simulink model "QuadArchitecture_AI"  (R2026b)
settings: Solver=ode4  StopTime=90  FixedStep=0.005
InitFcn:
  | init_stage02
settings Model: DataDictionary=QuadInterfaces_AI.sldd  Creator=JonathanTee  LastModifiedBy=JonathanTee

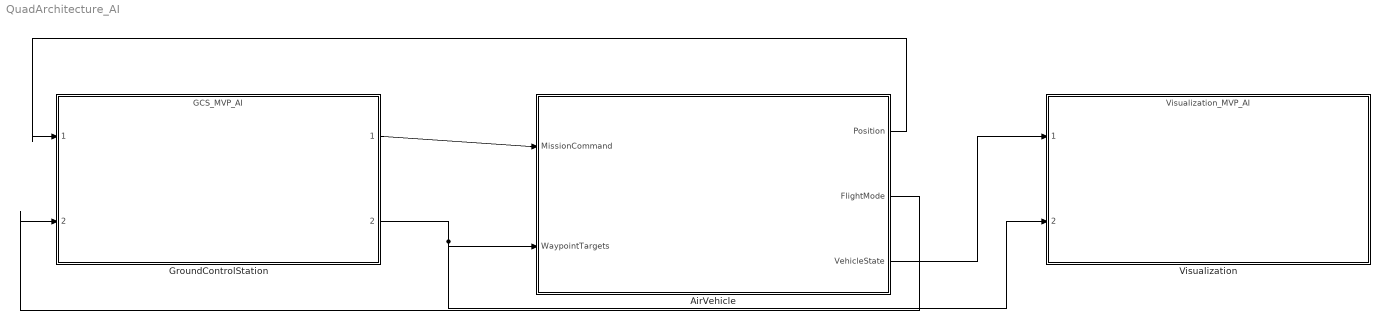
== system QuadArchitecture_AI ==
  AirVehicle : Subsystem
      settings: PortSchema="{\"entries\":[{\"content\":{\"headerSize\":26,\"margin\":15,\"minimumSpacing\":25,\"sides\":[{\"content\":{\"connectorIds\":[\"In1\",\"In2\"]},\"type\":\"ConnectorPlacement.EquallySpacedRectSide\",\"uuid\":\"ecfb2a5d-ebc3-4605-9a84-c6fd342510eb\"},{\"content\":{\"connectorIds\":[\"Out1\",\"Out2\",\"Out3\"],\"side\":\"RIGHT\"},\"type\":\"ConnectorPlacement.EquallySpacedRectSide\",\"uuid\":\"41ea779c-ccae-40c9-bf4c-62eb2a12d4ec\"},{\"content\":{\"side\":\"TOP\"},\"type\":\"ConnectorPlacement.EquallySpacedRectSide\",\"uuid\":\"f1fc56fa-babc-4d23-97d2-f02afcdd55d8\"}]},\"type\":\"ConnectorPlacement.EquallySpacedConnector\",\"uuid\":\"2007e49f-3d37-456e-85ff-e7f0d83353ae\"}],\"packageUris\":[\"http://schema.mathworks.com/mf0/Connector/R2020b\"],\"version\":\"1.0\"}"
  GroundControlStation : ModelReference  ModelNameDialog=GCS_MVP_AI  SimulationMode=Normal  ModelReferenceVersion=1.3
      settings: PortSchema="{\"entries\":[{\"content\":{\"headerSize\":38,\"margin\":15,\"minimumSpacing\":25,\"sides\":[{\"content\":{\"connectorIds\":[\"In1\",\"In2\"]},\"type\":\"ConnectorPlacement.EquallySpacedRectSide\",\"uuid\":\"ecfb2a5d-ebc3-4605-9a84-c6fd342510eb\"},{\"content\":{\"connectorIds\":[\"Out1\",\"Out2\"],\"side\":\"RIGHT\"},\"type\":\"ConnectorPlacement.EquallySpacedRectSide\",\"uuid\":\"41ea779c-ccae-40c9-bf4c-62eb2a12d4ec\"},{\"content\":{\"side\":\"TOP\"},\"type\":\"ConnectorPlacement.EquallySpacedRectSide\",\"uuid\":\"f1fc56fa-babc-4d23-97d2-f02afcdd55d8\"}]},\"type\":\"ConnectorPlacement.EquallySpacedConnector\",\"uuid\":\"2007e49f-3d37-456e-85ff-e7f0d83353ae\"}],\"packageUris\":[\"http://schema.mathworks.com/mf0/Connector/R2020b\"],\"version\":\"1.0\"}"
  Visualization : ModelReference  ModelNameDialog=Visualization_MVP_AI  SimulationMode=Normal  ModelReferenceVersion=1.2
      settings: PortSchema="{\"entries\":[{\"content\":{\"headerSize\":38,\"margin\":15,\"minimumSpacing\":25,\"sides\":[{\"content\":{\"connectorIds\":[\"In1\",\"In2\"]},\"type\":\"ConnectorPlacement.EquallySpacedRectSide\",\"uuid\":\"ecfb2a5d-ebc3-4605-9a84-c6fd342510eb\"},{\"content\":{\"side\":\"RIGHT\"},\"type\":\"ConnectorPlacement.EquallySpacedRectSide\",\"uuid\":\"41ea779c-ccae-40c9-bf4c-62eb2a12d4ec\"},{\"content\":{\"side\":\"TOP\"},\"type\":\"ConnectorPlacement.EquallySpacedRectSide\",\"uuid\":\"f1fc56fa-babc-4d23-97d2-f02afcdd55d8\"}]},\"type\":\"ConnectorPlacement.EquallySpacedConnector\",\"uuid\":\"2007e49f-3d37-456e-85ff-e7f0d83353ae\"}],\"packageUris\":[\"http://schema.mathworks.com/mf0/Connector/R2020b\"],\"version\":\"1.0\"}"
  wires:
  AirVehicle/2(FlightMode) -> GroundControlStation/2
  AirVehicle/1(Position) -> GroundControlStation/1
  GroundControlStation/1 -> AirVehicle/1(MissionCommand)
  GroundControlStation/2 -> AirVehicle/2(WaypointTargets), Visualization/2
  AirVehicle/3(VehicleState) -> Visualization/1

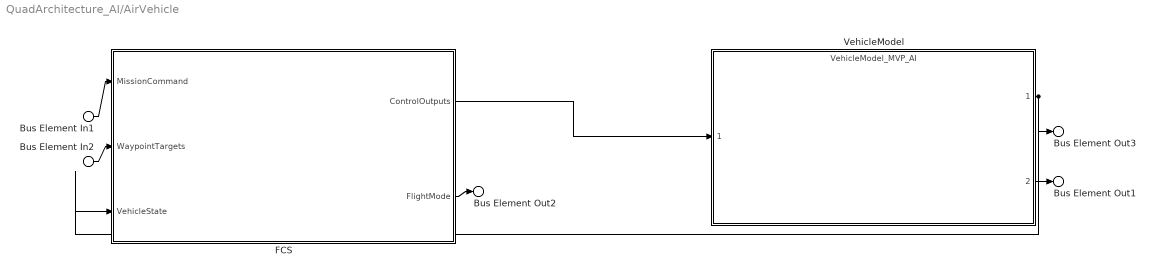
== system QuadArchitecture_AI/AirVehicle ==
  Bus Element In1 : Inport  PortName=MissionCommand
  Bus Element In2 : Inport  Port=2  PortName=WaypointTargets
  FCS : Subsystem
      settings: PortSchema="{\"entries\":[{\"content\":{\"headerSize\":26,\"margin\":15,\"minimumSpacing\":25,\"sides\":[{\"content\":{\"connectorIds\":[\"In1\",\"In2\",\"In3\"]},\"type\":\"ConnectorPlacement.EquallySpacedRectSide\",\"uuid\":\"ecfb2a5d-ebc3-4605-9a84-c6fd342510eb\"},{\"content\":{\"connectorIds\":[\"Out1\",\"Out2\"],\"side\":\"RIGHT\"},\"type\":\"ConnectorPlacement.EquallySpacedRectSide\",\"uuid\":\"41ea779c-ccae-40c9-bf4c-62eb2a12d4ec\"},{\"content\":{\"side\":\"TOP\"},\"type\":\"ConnectorPlacement.EquallySpacedRectSide\",\"uuid\":\"f1fc56fa-babc-4d23-97d2-f02afcdd55d8\"}]},\"type\":\"ConnectorPlacement.EquallySpacedConnector\",\"uuid\":\"2007e49f-3d37-456e-85ff-e7f0d83353ae\"}],\"packageUris\":[\"http://schema.mathworks.com/mf0/Connector/R2020b\"],\"version\":\"1.0\"}"
  VehicleModel : ModelReference  ModelNameDialog=VehicleModel_MVP_AI  SimulationMode=Normal  ModelReferenceVersion=1.4
      settings: PortSchema="{\"entries\":[{\"content\":{\"headerSize\":38,\"margin\":15,\"minimumSpacing\":25,\"sides\":[{\"content\":{\"connectorIds\":[\"In1\"]},\"type\":\"ConnectorPlacement.EquallySpacedRectSide\",\"uuid\":\"ecfb2a5d-ebc3-4605-9a84-c6fd342510eb\"},{\"content\":{\"connectorIds\":[\"Out1\",\"Out2\"],\"side\":\"RIGHT\"},\"type\":\"ConnectorPlacement.EquallySpacedRectSide\",\"uuid\":\"41ea779c-ccae-40c9-bf4c-62eb2a12d4ec\"},{\"content\":{\"side\":\"TOP\"},\"type\":\"ConnectorPlacement.EquallySpacedRectSide\",\"uuid\":\"f1fc56fa-babc-4d23-97d2-f02afcdd55d8\"}]},\"type\":\"ConnectorPlacement.EquallySpacedConnector\",\"uuid\":\"2007e49f-3d37-456e-85ff-e7f0d83353ae\"}],\"packageUris\":[\"http://schema.mathworks.com/mf0/Connector/R2020b\"],\"version\":\"1.0\"}"
  Bus Element Out1 : Outport  PortName=Position
  Bus Element Out2 : Outport  Port=2  PortName=FlightMode
  Bus Element Out3 : Outport  Port=3  PortName=VehicleState
  wires:
  FCS/2(FlightMode) -> Bus Element Out2/1
  Bus Element In2/1 -> FCS/2(WaypointTargets)
  Bus Element In1/1 -> FCS/1(MissionCommand)
  FCS/1(ControlOutputs) -> VehicleModel/1
  VehicleModel/2 -> Bus Element Out1/1
  VehicleModel/1 -> Bus Element Out3/1, FCS/3(VehicleState)

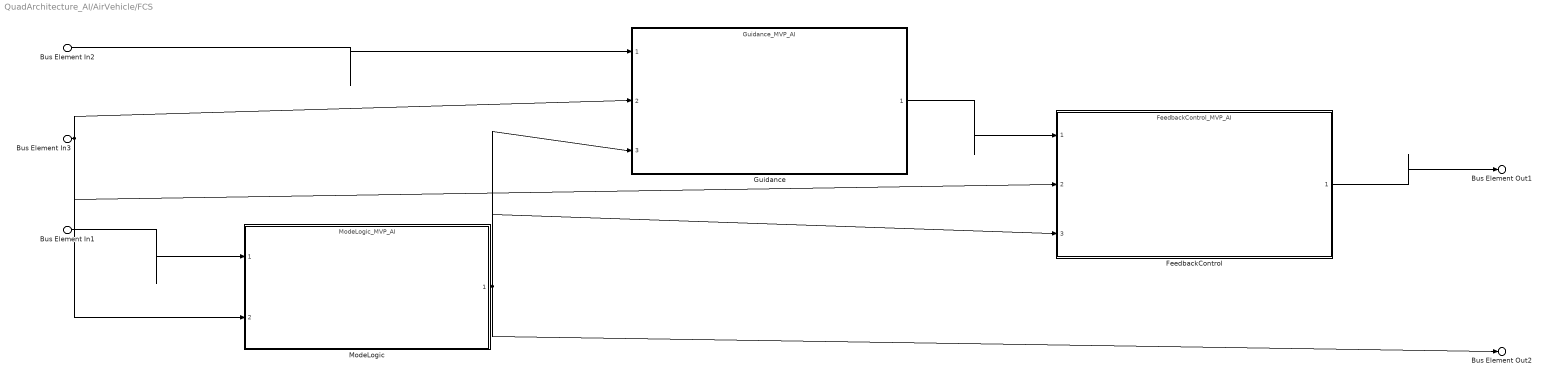
== system QuadArchitecture_AI/AirVehicle/FCS ==
  Bus Element In1 : Inport  PortName=MissionCommand
  Bus Element In2 : Inport  Port=2  PortName=WaypointTargets
  Bus Element In3 : Inport  Port=3  PortName=VehicleState
  FeedbackControl : ModelReference  ModelNameDialog=FeedbackControl_MVP_AI  SimulationMode=Normal  ModelReferenceVersion=1.3
      settings: PortSchema="{\"entries\":[{\"content\":{\"headerSize\":38,\"margin\":15,\"minimumSpacing\":25,\"sides\":[{\"content\":{\"connectorIds\":[\"In1\",\"In2\",\"In3\"]},\"type\":\"ConnectorPlacement.EquallySpacedRectSide\",\"uuid\":\"ecfb2a5d-ebc3-4605-9a84-c6fd342510eb\"},{\"content\":{\"connectorIds\":[\"Out1\"],\"side\":\"RIGHT\"},\"type\":\"ConnectorPlacement.EquallySpacedRectSide\",\"uuid\":\"41ea779c-ccae-40c9-bf4c-62eb2a12d4ec\"},{\"content\":{\"side\":\"TOP\"},\"type\":\"ConnectorPlacement.EquallySpacedRectSide\",\"uuid\":\"f1fc56fa-babc-4d23-97d2-f02afcdd55d8\"}]},\"type\":\"ConnectorPlacement.EquallySpacedConnector\",\"uuid\":\"2007e49f-3d37-456e-85ff-e7f0d83353ae\"}],\"packageUris\":[\"http://schema.mathworks.com/mf0/Connector/R2020b\"],\"version\":\"1.0\"}"
  Guidance : ModelReference  ModelNameDialog=Guidance_MVP_AI  SimulationMode=Normal  ModelReferenceVersion=1.2
      settings: PortSchema="{\"entries\":[{\"content\":{\"headerSize\":38,\"margin\":15,\"minimumSpacing\":25,\"sides\":[{\"content\":{\"connectorIds\":[\"In1\",\"In2\",\"In3\"]},\"type\":\"ConnectorPlacement.EquallySpacedRectSide\",\"uuid\":\"ecfb2a5d-ebc3-4605-9a84-c6fd342510eb\"},{\"content\":{\"connectorIds\":[\"Out1\"],\"side\":\"RIGHT\"},\"type\":\"ConnectorPlacement.EquallySpacedRectSide\",\"uuid\":\"41ea779c-ccae-40c9-bf4c-62eb2a12d4ec\"},{\"content\":{\"side\":\"TOP\"},\"type\":\"ConnectorPlacement.EquallySpacedRectSide\",\"uuid\":\"f1fc56fa-babc-4d23-97d2-f02afcdd55d8\"}]},\"type\":\"ConnectorPlacement.EquallySpacedConnector\",\"uuid\":\"2007e49f-3d37-456e-85ff-e7f0d83353ae\"}],\"packageUris\":[\"http://schema.mathworks.com/mf0/Connector/R2020b\"],\"version\":\"1.0\"}"
  ModeLogic : ModelReference  ModelNameDialog=ModeLogic_MVP_AI  SimulationMode=Normal  ModelReferenceVersion=1.2
      settings: PortSchema="{\"entries\":[{\"content\":{\"headerSize\":38,\"margin\":15,\"minimumSpacing\":25,\"sides\":[{\"content\":{\"connectorIds\":[\"In1\",\"In2\"]},\"type\":\"ConnectorPlacement.EquallySpacedRectSide\",\"uuid\":\"ecfb2a5d-ebc3-4605-9a84-c6fd342510eb\"},{\"content\":{\"connectorIds\":[\"Out1\"],\"side\":\"RIGHT\"},\"type\":\"ConnectorPlacement.EquallySpacedRectSide\",\"uuid\":\"41ea779c-ccae-40c9-bf4c-62eb2a12d4ec\"},{\"content\":{\"side\":\"TOP\"},\"type\":\"ConnectorPlacement.EquallySpacedRectSide\",\"uuid\":\"f1fc56fa-babc-4d23-97d2-f02afcdd55d8\"}]},\"type\":\"ConnectorPlacement.EquallySpacedConnector\",\"uuid\":\"2007e49f-3d37-456e-85ff-e7f0d83353ae\"}],\"packageUris\":[\"http://schema.mathworks.com/mf0/Connector/R2020b\"],\"version\":\"1.0\"}"
  Bus Element Out1 : Outport  PortName=ControlOutputs
  Bus Element Out2 : Outport  Port=2  PortName=FlightMode
  wires:
  Bus Element In3/1 -> ModeLogic/2, Guidance/2, FeedbackControl/2
  Bus Element In1/1 -> ModeLogic/1
  ModeLogic/1 -> Bus Element Out2/1, Guidance/3, FeedbackControl/3
  Bus Element In2/1 -> Guidance/1
  Guidance/1 -> FeedbackControl/1
  FeedbackControl/1 -> Bus Element Out1/1
